simulink library "Turbine_State_Machine_Lib"  (R2025a)
settings: Solver=ode45  StartTime=0.0  StopTime=10.0  RelTol=1e-3  EnableMultiTasking=on
Description:
  | Copyright 2009-2025 The MathWorks, Inc. MathWorks, Inc.
settings Model: Creator=smiller  LastModifiedBy=smiller
settings SolverCC: AlgebraicLoopSolver=TrustRegion
settings DataIOCC: LimitDataPoints=on  SaveFormat=Array  SignalLoggingSaveFormat=ModelDataLogs  ReturnWorkspaceOutputs=off
settings OptimizationCC: ReuseModelBlockBuffer=off  ExpressionDepthLimit=2147483647.0  LifeSpan=inf
settings DebuggingCC: UnderspecifiedInitializationDetection=Classic  MergeDetectMultiDrivingBlocksExec=none  SolverPrmCheckMsg=warning  FcnCallInpInsideContextMsg=warning  UnconnectedInputMsg=warning  UnconnectedOutputMsg=warning  UnconnectedLineMsg=warning  AllowSymbolicDim=off  StateNameClashWarn=warning  PregeneratedLibrarySubsystemCodeDiagnostic=none  SFUnexpectedBacktrackingDiag=warning  SFNoUnconditionalDefaultTransitionDiag=warning  SFExecutionAtInitializationDiag=none  ArithmeticOperatorsInVariantConditions=warning
settings HardwareCC: ProdBitPerPointer=32.0  ProdBitPerSizeT=32.0  ProdBitPerPtrDiffT=32.0  ProdLargestAtomicFloat=None  ProdIntDivRoundTo=Undefined  ProdEndianess=Unspecified  ProdWordSize=32.0  ProdHWDeviceType=32-bit Generic
settings ModelReferenceCC: EnableRefExpFcnMdlSchedulingChecks=on  PropagateSignalLabelsOutOfModel=off
settings SFSimCC: SimUseLocalCustomCode=off  CustomCodeUndefinedFunction=UseInterfaceOnly
settings RTWCC: RTWUseLocalCustomCode=off  GPUComputeCapability=3.5  DLArmComputeVersion=19.05
settings CodeAppCC: StateflowObjectComments=on
settings GRTTargetCC: TargetLangStandard=C89/C90 (ANSI)  CombineOutputUpdateFcns=off  GRTInterface=on
settings ConfigComp: CovMetricSettings=dw  CovSaveCumulativeToWorkspaceVar=on  CovSaveSingleToWorkspaceVar=on  CovExternalEMLEnable=off  CovSFcnEnable=off

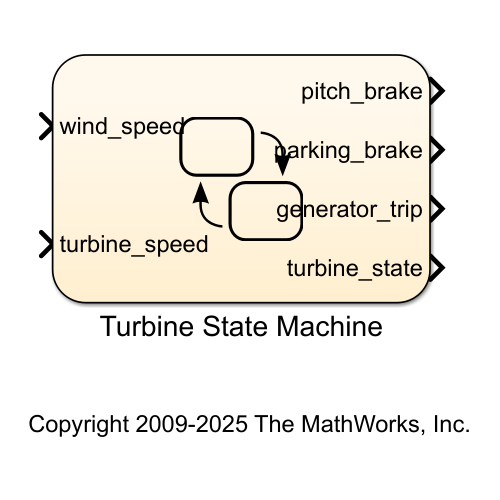
[thumbnail: Simulink's stored preview of the top-level diagram]
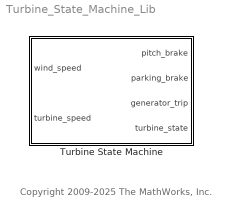
== system Turbine_State_Machine_Lib ==
  note: Copyright 2009-2025 The MathWorks, Inc.
  Turbine State Machine : Stateflow chart  TreatAsAtomicUnit=on

== stateflow chart Turbine_State_Machine_Lib/Turbine State Machine ==
  state Generating
    entry: parking_brake = 0;
    generator_trip = 0;
    pitch_brake = 0;
    turbine_state = 2;
  state Startup
    entry: parking_brake = 0;
    generator_trip = 1;
    pitch_brake = 0;
    turbine_state = 1;
  state Park
    entry: parking_brake = 1;
    generator_trip = 1;
    pitch_brake = 1;
    turbine_state = 0;
  state Brake
    entry: parking_brake = 0;
    generator_trip = 1;
    pitch_brake = 1;
    turbine_state = 3;
  Startup -> Generating [order 1] : [turbine_speed>...
      | turbine_speed_cut_in]
  Park -> Startup : [wind_speed>...
      | wind_speed_cut_in_lower...
      | &&wind_speed<...
      | wind_speed_cut_out]
  Startup -> Brake [order 2] : [wind_speed<...
      | wind_speed_cut_in_lower]
  Brake -> Startup [order 2] : [wind_speed<...
      | wind_speed_cut_in_upper...
      | && wind_speed>...
      | wind_speed_cut_in_lower]
  Generating -> Brake : [wind_speed<...
      | wind_speed_cut_in_lower...
      | ||wind_speed>...
      | wind_speed_cut_out...
      | ||turbine_speed>...
      | turbine_speed_cut_out...
      | ||turbine_speed<...
      | turbine_speed_cut_in*0.9]
  (default) -> Park
  Brake -> Park [order 1] : [turbine_speed<=...
      | park_speed]
  data: pitch_brake output double; wind_speed input; turbine_speed input; parking_brake output double; generator_trip output double; wind_speed_cut_in_lower local double =WT_Params.Main_Controller.wind_speed_cut_in_lower; turbine_speed_cut_in local double =WT_Params.Main_Controller.turbine_speed_cut_in; turbine_state output double; wind_speed_cut_out local double =WT_Params.Main_Controller.wind_speed_cut_out; wind_speed_cut_in_upper local double =WT_Params.Main_Controller.wind_speed_cut_in_upper; turbine_speed_cut_out local double =WT_Params.Main_Controller.turbine_speed_cut_out; park_speed constant double =WT_Params.Main_Controller.turbine_speed_park
